simulink model "pi_rotation_loss"  (R2025b)
settings: Solver=VariableStepAuto  StartTime=0.0  StopTime=10.0  RelTol=1e-3
undefined symbols (not defined in the file): Eoff_mJ, Eon_mJ, Ic_bp, Ic_bp1, Ion, Lithium, Vce_bp
libraries: spsCurrentMeasurementLib x19, spsMosfetLib x16, simulink x16, hdlsllib x16, spsSeriesRLCBranchLib x14, spsVoltageMeasurementLib x5, spsBatteryLib x2, spsLinearTransformerLib x1, slpidlib x1, spspowerguiLib x1
(part 2 of 2)

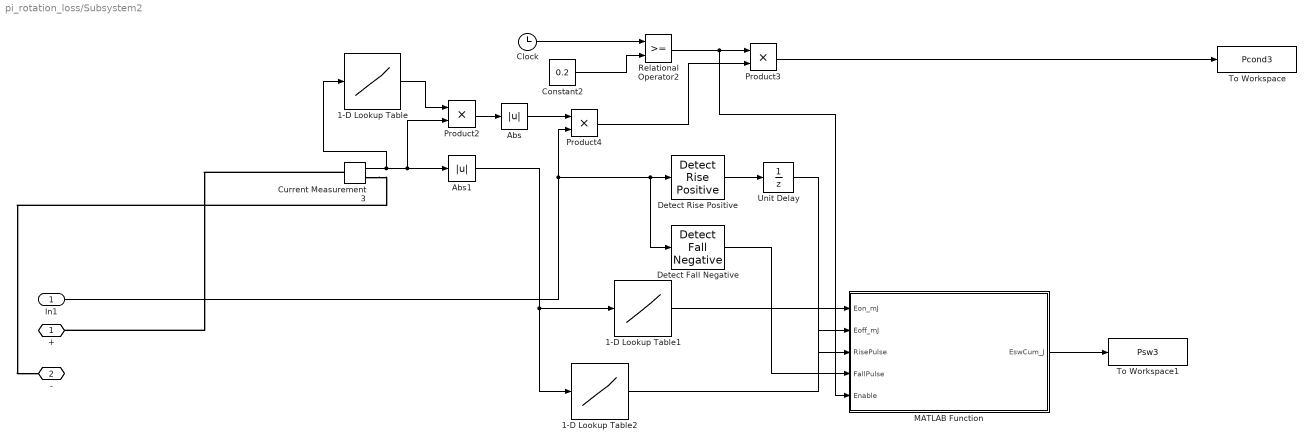
== system pi_rotation_loss/Subsystem2 ==
  In1 : Inport
  1-D Lookup Table : Lookup_n-D  NumberOfTableDimensions=1  BreakpointsForDimension1=Ic_bp  Table=Vce_bp  InternalRulePriority=Speed  RndMeth=Simplest
  1-D Lookup Table1 : Lookup_n-D  NumberOfTableDimensions=1  BreakpointsForDimension1=Ic_bp1  Table=Eon_mJ  InternalRulePriority=Speed  RndMeth=Simplest
  1-D Lookup Table2 : Lookup_n-D  NumberOfTableDimensions=1  BreakpointsForDimension1=Ic_bp1  Table=Eoff_mJ  InternalRulePriority=Speed  RndMeth=Simplest
  Abs : Abs  SaturateOnIntegerOverflow=off
  Abs1 : Abs  SaturateOnIntegerOverflow=off
  Clock : Clock
  Constant2 : Constant  Value=0.2
  Current Measurement3 : spsCurrentMeasurementLib/Current Measurement  PhasorSimulation=off  OutputType=Complex  PSBequivalent=0
  Detect Fall Negative : simulink/Logic and Bit Operations/Detect Fall Negative  vinit=0  OutDataTypeStr=boolean
  Detect Rise Positive : hdlsllib/Logic and Bit Operations/Detect Rise Positive  vinit=0  OutDataTypeStr=boolean
  MATLAB Function : MATLAB Function  TreatAsAtomicUnit=on
  Product2 : Product
  Product3 : Product
  Product4 : Product
  Relational Operator2 : RelationalOperator  OutDataTypeStr=boolean  RndMeth=Simplest  InputSameDT=off
  To Workspace : ToWorkspace  VariableName=Pcond3  SaveFormat=Timeseries  SampleTime=-1
  To Workspace1 : ToWorkspace  VariableName=Psw3  SaveFormat=Timeseries  SampleTime=-1
  Unit Delay : UnitDelay  SampleTime=-1  HasFrameUpgradeWarning=on
  + : PMIOPort  Side=Left
  - : PMIOPort  Port=2  Side=Right
  wires:
  Clock/1 -> Relational Operator2/1
  Abs/1 -> Product4/1
  Current Measurement3/1 -> Product2/2, Abs1/1, 1-D Lookup Table/1
  Unit Delay/1 -> MATLAB Function/3(RisePulse)
  1-D Lookup Table1/1 -> MATLAB Function/1(Eon_mJ)
  In1/1 -> Product4/2, Detect Fall Negative/1, Detect Rise Positive/1
  Product3/1 -> To Workspace/1
  Detect Rise Positive/1 -> Unit Delay/1
  Relational Operator2/1 -> MATLAB Function/5(Enable), Product3/1
  Product4/1 -> Product3/2
  Product2/1 -> Abs/1
  MATLAB Function/1(EswCum_J) -> To Workspace1/1
  1-D Lookup Table2/1 -> MATLAB Function/2(Eoff_mJ)
  Constant2/1 -> Relational Operator2/2
  Detect Fall Negative/1 -> MATLAB Function/4(FallPulse)
  1-D Lookup Table/1 -> Product2/1
  Abs1/1 -> 1-D Lookup Table2/1, 1-D Lookup Table1/1
  connections:
  Current Measurement3/LConn1 -- +/RConn1
  Current Measurement3/RConn1 -- -/RConn1

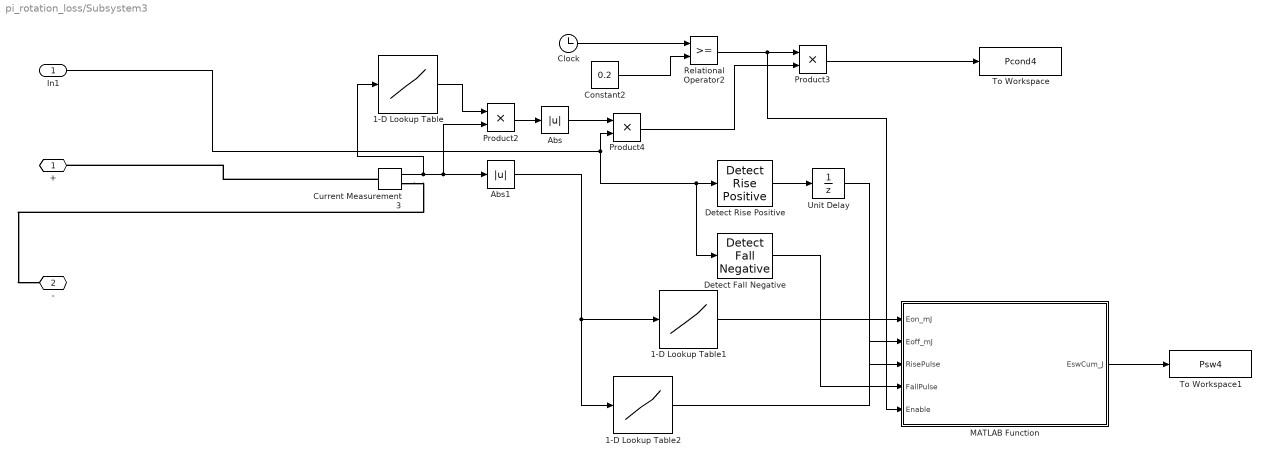
== system pi_rotation_loss/Subsystem3 ==
  In1 : Inport
  1-D Lookup Table : Lookup_n-D  NumberOfTableDimensions=1  BreakpointsForDimension1=Ic_bp  Table=Vce_bp  InternalRulePriority=Speed  RndMeth=Simplest
  1-D Lookup Table1 : Lookup_n-D  NumberOfTableDimensions=1  BreakpointsForDimension1=Ic_bp1  Table=Eon_mJ  InternalRulePriority=Speed  RndMeth=Simplest
  1-D Lookup Table2 : Lookup_n-D  NumberOfTableDimensions=1  BreakpointsForDimension1=Ic_bp1  Table=Eoff_mJ  InternalRulePriority=Speed  RndMeth=Simplest
  Abs : Abs  SaturateOnIntegerOverflow=off
  Abs1 : Abs  SaturateOnIntegerOverflow=off
  Clock : Clock
  Constant2 : Constant  Value=0.2
  Current Measurement3 : spsCurrentMeasurementLib/Current Measurement  PhasorSimulation=off  OutputType=Complex  PSBequivalent=0
  Detect Fall Negative : simulink/Logic and Bit Operations/Detect Fall Negative  vinit=0  OutDataTypeStr=boolean
  Detect Rise Positive : hdlsllib/Logic and Bit Operations/Detect Rise Positive  vinit=0  OutDataTypeStr=boolean
  MATLAB Function : MATLAB Function  TreatAsAtomicUnit=on
  Product2 : Product
  Product3 : Product
  Product4 : Product
  Relational Operator2 : RelationalOperator  OutDataTypeStr=boolean  RndMeth=Simplest  InputSameDT=off
  To Workspace : ToWorkspace  VariableName=Pcond4  SaveFormat=Timeseries  SampleTime=-1
  To Workspace1 : ToWorkspace  VariableName=Psw4  SaveFormat=Timeseries  SampleTime=-1
  Unit Delay : UnitDelay  SampleTime=-1  HasFrameUpgradeWarning=on
  + : PMIOPort  Side=Left
  - : PMIOPort  Port=2  Side=Right
  wires:
  Clock/1 -> Relational Operator2/1
  Abs/1 -> Product4/1
  Current Measurement3/1 -> Product2/2, Abs1/1, 1-D Lookup Table/1
  Unit Delay/1 -> MATLAB Function/3(RisePulse)
  1-D Lookup Table1/1 -> MATLAB Function/1(Eon_mJ)
  In1/1 -> Product4/2, Detect Fall Negative/1, Detect Rise Positive/1
  Product3/1 -> To Workspace/1
  Detect Rise Positive/1 -> Unit Delay/1
  Relational Operator2/1 -> MATLAB Function/5(Enable), Product3/1
  Product4/1 -> Product3/2
  Product2/1 -> Abs/1
  MATLAB Function/1(EswCum_J) -> To Workspace1/1
  1-D Lookup Table2/1 -> MATLAB Function/2(Eoff_mJ)
  Constant2/1 -> Relational Operator2/2
  Detect Fall Negative/1 -> MATLAB Function/4(FallPulse)
  1-D Lookup Table/1 -> Product2/1
  Abs1/1 -> 1-D Lookup Table2/1, 1-D Lookup Table1/1
  connections:
  Current Measurement3/LConn1 -- +/RConn1
  Current Measurement3/RConn1 -- -/RConn1

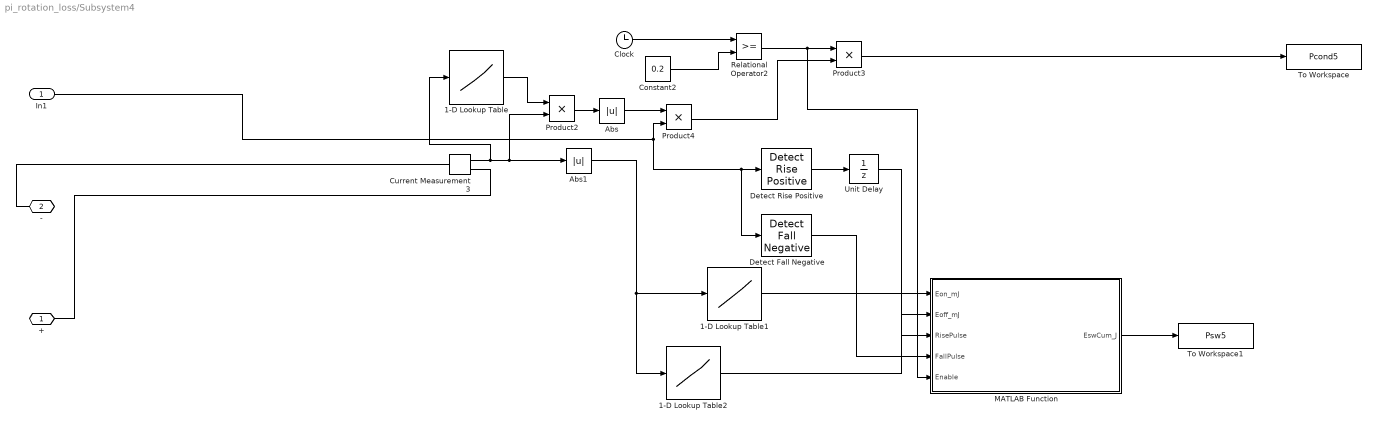
== system pi_rotation_loss/Subsystem4 ==
  In1 : Inport
  1-D Lookup Table : Lookup_n-D  NumberOfTableDimensions=1  BreakpointsForDimension1=Ic_bp  Table=Vce_bp  InternalRulePriority=Speed  RndMeth=Simplest
  1-D Lookup Table1 : Lookup_n-D  NumberOfTableDimensions=1  BreakpointsForDimension1=Ic_bp1  Table=Eon_mJ  InternalRulePriority=Speed  RndMeth=Simplest
  1-D Lookup Table2 : Lookup_n-D  NumberOfTableDimensions=1  BreakpointsForDimension1=Ic_bp1  Table=Eoff_mJ  InternalRulePriority=Speed  RndMeth=Simplest
  Abs : Abs  SaturateOnIntegerOverflow=off
  Abs1 : Abs  SaturateOnIntegerOverflow=off
  Clock : Clock
  Constant2 : Constant  Value=0.2
  Current Measurement3 : spsCurrentMeasurementLib/Current Measurement  PhasorSimulation=off  OutputType=Complex  PSBequivalent=0
  Detect Fall Negative : simulink/Logic and Bit Operations/Detect Fall Negative  vinit=0  OutDataTypeStr=boolean
  Detect Rise Positive : hdlsllib/Logic and Bit Operations/Detect Rise Positive  vinit=0  OutDataTypeStr=boolean
  MATLAB Function : MATLAB Function  TreatAsAtomicUnit=on
  Product2 : Product
  Product3 : Product
  Product4 : Product
  Relational Operator2 : RelationalOperator  OutDataTypeStr=boolean  RndMeth=Simplest  InputSameDT=off
  To Workspace : ToWorkspace  VariableName=Pcond5  SaveFormat=Timeseries  SampleTime=-1
  To Workspace1 : ToWorkspace  VariableName=Psw5  SaveFormat=Timeseries  SampleTime=-1
  Unit Delay : UnitDelay  SampleTime=-1  HasFrameUpgradeWarning=on
  + : PMIOPort  Side=Left
  - : PMIOPort  Port=2  Side=Right
  wires:
  Clock/1 -> Relational Operator2/1
  Abs/1 -> Product4/1
  Current Measurement3/1 -> Product2/2, Abs1/1, 1-D Lookup Table/1
  Unit Delay/1 -> MATLAB Function/3(RisePulse)
  1-D Lookup Table1/1 -> MATLAB Function/1(Eon_mJ)
  In1/1 -> Product4/2, Detect Fall Negative/1, Detect Rise Positive/1
  Product3/1 -> To Workspace/1
  Detect Rise Positive/1 -> Unit Delay/1
  Relational Operator2/1 -> MATLAB Function/5(Enable), Product3/1
  Product4/1 -> Product3/2
  Product2/1 -> Abs/1
  MATLAB Function/1(EswCum_J) -> To Workspace1/1
  1-D Lookup Table2/1 -> MATLAB Function/2(Eoff_mJ)
  Constant2/1 -> Relational Operator2/2
  Detect Fall Negative/1 -> MATLAB Function/4(FallPulse)
  1-D Lookup Table/1 -> Product2/1
  Abs1/1 -> 1-D Lookup Table2/1, 1-D Lookup Table1/1
  connections:
  Current Measurement3/LConn1 -- -/RConn1
  Current Measurement3/RConn1 -- +/RConn1

== system pi_rotation_loss/Subsystem5 ==
  In1 : Inport
  1-D Lookup Table : Lookup_n-D  NumberOfTableDimensions=1  BreakpointsForDimension1=Ic_bp  Table=Vce_bp  InternalRulePriority=Speed  RndMeth=Simplest
  1-D Lookup Table1 : Lookup_n-D  NumberOfTableDimensions=1  BreakpointsForDimension1=Ic_bp1  Table=Eon_mJ  InternalRulePriority=Speed  RndMeth=Simplest
  1-D Lookup Table2 : Lookup_n-D  NumberOfTableDimensions=1  BreakpointsForDimension1=Ic_bp1  Table=Eoff_mJ  InternalRulePriority=Speed  RndMeth=Simplest
  Abs : Abs  SaturateOnIntegerOverflow=off
  Abs1 : Abs  SaturateOnIntegerOverflow=off
  Clock : Clock
  Constant2 : Constant  Value=0.2
  Current Measurement3 : spsCurrentMeasurementLib/Current Measurement  PhasorSimulation=off  OutputType=Complex  PSBequivalent=0
  Detect Fall Negative : simulink/Logic and Bit Operations/Detect Fall Negative  vinit=0  OutDataTypeStr=boolean
  Detect Rise Positive : hdlsllib/Logic and Bit Operations/Detect Rise Positive  vinit=0  OutDataTypeStr=boolean
  MATLAB Function : MATLAB Function  TreatAsAtomicUnit=on
  Product2 : Product
  Product3 : Product
  Product4 : Product
  Relational Operator2 : RelationalOperator  OutDataTypeStr=boolean  RndMeth=Simplest  InputSameDT=off
  To Workspace : ToWorkspace  VariableName=Pcond6  SaveFormat=Timeseries  SampleTime=-1
  To Workspace1 : ToWorkspace  VariableName=Psw6  SaveFormat=Timeseries  SampleTime=-1
  Unit Delay : UnitDelay  SampleTime=-1  HasFrameUpgradeWarning=on
  + : PMIOPort  Side=Left
  - : PMIOPort  Port=2  Side=Right
  wires:
  Clock/1 -> Relational Operator2/1
  Abs/1 -> Product4/1
  Current Measurement3/1 -> Product2/2, Abs1/1, 1-D Lookup Table/1
  Unit Delay/1 -> MATLAB Function/3(RisePulse)
  1-D Lookup Table1/1 -> MATLAB Function/1(Eon_mJ)
  In1/1 -> Product4/2, Detect Fall Negative/1, Detect Rise Positive/1
  Product3/1 -> To Workspace/1
  Detect Rise Positive/1 -> Unit Delay/1
  Relational Operator2/1 -> MATLAB Function/5(Enable), Product3/1
  Product4/1 -> Product3/2
  Product2/1 -> Abs/1
  MATLAB Function/1(EswCum_J) -> To Workspace1/1
  1-D Lookup Table2/1 -> MATLAB Function/2(Eoff_mJ)
  Constant2/1 -> Relational Operator2/2
  Detect Fall Negative/1 -> MATLAB Function/4(FallPulse)
  1-D Lookup Table/1 -> Product2/1
  Abs1/1 -> 1-D Lookup Table2/1, 1-D Lookup Table1/1
  connections:
  Current Measurement3/LConn1 -- +/RConn1
  Current Measurement3/RConn1 -- -/RConn1

== system pi_rotation_loss/Subsystem6 ==
  In1 : Inport
  1-D Lookup Table : Lookup_n-D  NumberOfTableDimensions=1  BreakpointsForDimension1=Ic_bp  Table=Vce_bp  InternalRulePriority=Speed  RndMeth=Simplest
  1-D Lookup Table1 : Lookup_n-D  NumberOfTableDimensions=1  BreakpointsForDimension1=Ic_bp1  Table=Eon_mJ  InternalRulePriority=Speed  RndMeth=Simplest
  1-D Lookup Table2 : Lookup_n-D  NumberOfTableDimensions=1  BreakpointsForDimension1=Ic_bp1  Table=Eoff_mJ  InternalRulePriority=Speed  RndMeth=Simplest
  Abs : Abs  SaturateOnIntegerOverflow=off
  Abs1 : Abs  SaturateOnIntegerOverflow=off
  Clock : Clock
  Constant2 : Constant  Value=0.2
  Current Measurement3 : spsCurrentMeasurementLib/Current Measurement  PhasorSimulation=off  OutputType=Complex  PSBequivalent=0
  Detect Fall Negative : simulink/Logic and Bit Operations/Detect Fall Negative  vinit=0  OutDataTypeStr=boolean
  Detect Rise Positive : hdlsllib/Logic and Bit Operations/Detect Rise Positive  vinit=0  OutDataTypeStr=boolean
  MATLAB Function : MATLAB Function  TreatAsAtomicUnit=on
  Product2 : Product
  Product3 : Product
  Product4 : Product
  Relational Operator2 : RelationalOperator  OutDataTypeStr=boolean  RndMeth=Simplest  InputSameDT=off
  To Workspace : ToWorkspace  VariableName=Pcond8  SaveFormat=Timeseries  SampleTime=-1
  To Workspace1 : ToWorkspace  VariableName=Psw8  SaveFormat=Timeseries  SampleTime=-1
  Unit Delay : UnitDelay  SampleTime=-1  HasFrameUpgradeWarning=on
  + : PMIOPort  Side=Left
  - : PMIOPort  Port=2  Side=Right
  wires:
  Clock/1 -> Relational Operator2/1
  Abs/1 -> Product4/1
  Current Measurement3/1 -> Product2/2, Abs1/1, 1-D Lookup Table/1
  Unit Delay/1 -> MATLAB Function/3(RisePulse)
  1-D Lookup Table1/1 -> MATLAB Function/1(Eon_mJ)
  In1/1 -> Product4/2, Detect Fall Negative/1, Detect Rise Positive/1
  Product3/1 -> To Workspace/1
  Detect Rise Positive/1 -> Unit Delay/1
  Relational Operator2/1 -> MATLAB Function/5(Enable), Product3/1
  Product4/1 -> Product3/2
  Product2/1 -> Abs/1
  MATLAB Function/1(EswCum_J) -> To Workspace1/1
  1-D Lookup Table2/1 -> MATLAB Function/2(Eoff_mJ)
  Constant2/1 -> Relational Operator2/2
  Detect Fall Negative/1 -> MATLAB Function/4(FallPulse)
  1-D Lookup Table/1 -> Product2/1
  Abs1/1 -> 1-D Lookup Table2/1, 1-D Lookup Table1/1
  connections:
  Current Measurement3/LConn1 -- +/RConn1
  Current Measurement3/RConn1 -- -/RConn1

== system pi_rotation_loss/Subsystem7 ==
  In1 : Inport
  1-D Lookup Table : Lookup_n-D  NumberOfTableDimensions=1  BreakpointsForDimension1=Ic_bp  Table=Vce_bp  InternalRulePriority=Speed  RndMeth=Simplest
  1-D Lookup Table1 : Lookup_n-D  NumberOfTableDimensions=1  BreakpointsForDimension1=Ic_bp1  Table=Eon_mJ  InternalRulePriority=Speed  RndMeth=Simplest
  1-D Lookup Table2 : Lookup_n-D  NumberOfTableDimensions=1  BreakpointsForDimension1=Ic_bp1  Table=Eoff_mJ  InternalRulePriority=Speed  RndMeth=Simplest
  Abs : Abs  SaturateOnIntegerOverflow=off
  Abs1 : Abs  SaturateOnIntegerOverflow=off
  Clock : Clock
  Constant2 : Constant  Value=0.2
  Current Measurement3 : spsCurrentMeasurementLib/Current Measurement  PhasorSimulation=off  OutputType=Complex  PSBequivalent=0
  Detect Fall Negative : simulink/Logic and Bit Operations/Detect Fall Negative  vinit=0  OutDataTypeStr=boolean
  Detect Rise Positive : hdlsllib/Logic and Bit Operations/Detect Rise Positive  vinit=0  OutDataTypeStr=boolean
  MATLAB Function : MATLAB Function  TreatAsAtomicUnit=on
  Product2 : Product
  Product3 : Product
  Product4 : Product
  Relational Operator2 : RelationalOperator  OutDataTypeStr=boolean  RndMeth=Simplest  InputSameDT=off
  To Workspace : ToWorkspace  VariableName=Pcond7  SaveFormat=Timeseries  SampleTime=-1
  To Workspace1 : ToWorkspace  VariableName=Psw7  SaveFormat=Timeseries  SampleTime=-1
  Unit Delay : UnitDelay  SampleTime=-1  HasFrameUpgradeWarning=on
  + : PMIOPort  Side=Left
  - : PMIOPort  Port=2  Side=Right
  wires:
  Clock/1 -> Relational Operator2/1
  Abs/1 -> Product4/1
  Current Measurement3/1 -> Product2/2, Abs1/1, 1-D Lookup Table/1
  Unit Delay/1 -> MATLAB Function/3(RisePulse)
  1-D Lookup Table1/1 -> MATLAB Function/1(Eon_mJ)
  In1/1 -> Product4/2, Detect Fall Negative/1, Detect Rise Positive/1
  Product3/1 -> To Workspace/1
  Detect Rise Positive/1 -> Unit Delay/1
  Relational Operator2/1 -> MATLAB Function/5(Enable), Product3/1
  Product4/1 -> Product3/2
  Product2/1 -> Abs/1
  MATLAB Function/1(EswCum_J) -> To Workspace1/1
  1-D Lookup Table2/1 -> MATLAB Function/2(Eoff_mJ)
  Constant2/1 -> Relational Operator2/2
  Detect Fall Negative/1 -> MATLAB Function/4(FallPulse)
  1-D Lookup Table/1 -> Product2/1
  Abs1/1 -> 1-D Lookup Table2/1, 1-D Lookup Table1/1
  connections:
  Current Measurement3/LConn1 -- +/RConn1
  Current Measurement3/RConn1 -- -/RConn1

== system pi_rotation_loss/Subsystem8 ==
  In1 : Inport
  1-D Lookup Table : Lookup_n-D  NumberOfTableDimensions=1  BreakpointsForDimension1=Ic_bp  Table=Vce_bp  InternalRulePriority=Speed  RndMeth=Simplest
  1-D Lookup Table1 : Lookup_n-D  NumberOfTableDimensions=1  BreakpointsForDimension1=Ic_bp1  Table=Eon_mJ  InternalRulePriority=Speed  RndMeth=Simplest
  1-D Lookup Table2 : Lookup_n-D  NumberOfTableDimensions=1  BreakpointsForDimension1=Ic_bp1  Table=Eoff_mJ  InternalRulePriority=Speed  RndMeth=Simplest
  Abs : Abs  SaturateOnIntegerOverflow=off
  Abs1 : Abs  SaturateOnIntegerOverflow=off
  Clock : Clock
  Constant2 : Constant  Value=0.2
  Current Measurement3 : spsCurrentMeasurementLib/Current Measurement  PhasorSimulation=off  OutputType=Complex  PSBequivalent=0
  Detect Fall Negative : simulink/Logic and Bit Operations/Detect Fall Negative  vinit=0  OutDataTypeStr=boolean
  Detect Rise Positive : hdlsllib/Logic and Bit Operations/Detect Rise Positive  vinit=0  OutDataTypeStr=boolean
  MATLAB Function : MATLAB Function  TreatAsAtomicUnit=on
  Product2 : Product
  Product3 : Product
  Product4 : Product
  Relational Operator2 : RelationalOperator  OutDataTypeStr=boolean  RndMeth=Simplest  InputSameDT=off
  To Workspace : ToWorkspace  VariableName=Pcond7_2  SaveFormat=Timeseries  SampleTime=-1
  To Workspace1 : ToWorkspace  VariableName=Psw7_2  SaveFormat=Timeseries  SampleTime=-1
  Unit Delay : UnitDelay  SampleTime=-1  HasFrameUpgradeWarning=on
  + : PMIOPort  Side=Left
  - : PMIOPort  Port=2  Side=Right
  wires:
  Clock/1 -> Relational Operator2/1
  Abs/1 -> Product4/1
  Current Measurement3/1 -> Product2/2, Abs1/1, 1-D Lookup Table/1
  Unit Delay/1 -> MATLAB Function/3(RisePulse)
  1-D Lookup Table1/1 -> MATLAB Function/1(Eon_mJ)
  In1/1 -> Product4/2, Detect Fall Negative/1, Detect Rise Positive/1
  Product3/1 -> To Workspace/1
  Detect Rise Positive/1 -> Unit Delay/1
  Relational Operator2/1 -> MATLAB Function/5(Enable), Product3/1
  Product4/1 -> Product3/2
  Product2/1 -> Abs/1
  MATLAB Function/1(EswCum_J) -> To Workspace1/1
  1-D Lookup Table2/1 -> MATLAB Function/2(Eoff_mJ)
  Constant2/1 -> Relational Operator2/2
  Detect Fall Negative/1 -> MATLAB Function/4(FallPulse)
  1-D Lookup Table/1 -> Product2/1
  Abs1/1 -> 1-D Lookup Table2/1, 1-D Lookup Table1/1
  connections:
  Current Measurement3/LConn1 -- +/RConn1
  Current Measurement3/RConn1 -- -/RConn1

== system pi_rotation_loss/Subsystem9 ==
  In1 : Inport
  1-D Lookup Table : Lookup_n-D  NumberOfTableDimensions=1  BreakpointsForDimension1=Ic_bp  Table=Vce_bp  InternalRulePriority=Speed  RndMeth=Simplest
  1-D Lookup Table1 : Lookup_n-D  NumberOfTableDimensions=1  BreakpointsForDimension1=Ic_bp1  Table=Eon_mJ  InternalRulePriority=Speed  RndMeth=Simplest
  1-D Lookup Table2 : Lookup_n-D  NumberOfTableDimensions=1  BreakpointsForDimension1=Ic_bp1  Table=Eoff_mJ  InternalRulePriority=Speed  RndMeth=Simplest
  Abs : Abs  SaturateOnIntegerOverflow=off
  Abs1 : Abs  SaturateOnIntegerOverflow=off
  Clock : Clock
  Constant2 : Constant  Value=0.2
  Current Measurement3 : spsCurrentMeasurementLib/Current Measurement  PhasorSimulation=off  OutputType=Complex  PSBequivalent=0
  Detect Fall Negative : simulink/Logic and Bit Operations/Detect Fall Negative  vinit=0  OutDataTypeStr=boolean
  Detect Rise Positive : hdlsllib/Logic and Bit Operations/Detect Rise Positive  vinit=0  OutDataTypeStr=boolean
  MATLAB Function : MATLAB Function  TreatAsAtomicUnit=on
  Product2 : Product
  Product3 : Product
  Product4 : Product
  Relational Operator2 : RelationalOperator  OutDataTypeStr=boolean  RndMeth=Simplest  InputSameDT=off
  To Workspace : ToWorkspace  VariableName=Pcond8_2  SaveFormat=Timeseries  SampleTime=-1
  To Workspace1 : ToWorkspace  VariableName=Psw8_2  SaveFormat=Timeseries  SampleTime=-1
  Unit Delay : UnitDelay  SampleTime=-1  HasFrameUpgradeWarning=on
  + : PMIOPort  Side=Left
  - : PMIOPort  Port=2  Side=Right
  wires:
  Clock/1 -> Relational Operator2/1
  Abs/1 -> Product4/1
  Current Measurement3/1 -> Product2/2, Abs1/1, 1-D Lookup Table/1
  Unit Delay/1 -> MATLAB Function/3(RisePulse)
  1-D Lookup Table1/1 -> MATLAB Function/1(Eon_mJ)
  In1/1 -> Product4/2, Detect Fall Negative/1, Detect Rise Positive/1
  Product3/1 -> To Workspace/1
  Detect Rise Positive/1 -> Unit Delay/1
  Relational Operator2/1 -> MATLAB Function/5(Enable), Product3/1
  Product4/1 -> Product3/2
  Product2/1 -> Abs/1
  MATLAB Function/1(EswCum_J) -> To Workspace1/1
  1-D Lookup Table2/1 -> MATLAB Function/2(Eoff_mJ)
  Constant2/1 -> Relational Operator2/2
  Detect Fall Negative/1 -> MATLAB Function/4(FallPulse)
  1-D Lookup Table/1 -> Product2/1
  Abs1/1 -> 1-D Lookup Table2/1, 1-D Lookup Table1/1
  connections:
  Current Measurement3/LConn1 -- +/RConn1
  Current Measurement3/RConn1 -- -/RConn1

== matlab function pi_rotation_loss/Subsystem15/MATLAB Function ==
  data: Eon_mJ input; EswCum_J output; Eoff_mJ input; RisePulse input; FallPulse input; Enable input
function EswCum_J = accumulate_energy( ...
    Eon_mJ, Eoff_mJ, RisePulse, FallPulse, Enable)
%#codegen
% Eon_mJ and Eoff_mJ are lookup outputs in millijoules.
% Output EswCum_J is cumulative switching energy in joules.
% Accumulate only events occurring after t = 0.2 s.

persistent cumulative_J

if isempty(cumulative_J)
    cumulative_J = 0.0;
end

if Enable > 0.5

    if RisePulse > 0.5
        cumulative_J = cumulative_J + max(Eon_mJ, 0) * 1e-3;
    end

    if FallPulse > 0.5
        cumulative_J = cumulative_J + max(Eoff_mJ, 0) * 1e-3;
    end

end

EswCum_J = cumulative_J;
end

== matlab function pi_rotation_loss/Subsystem/MATLAB Function ==
  data: Eon_mJ input; EswCum_J output; Eoff_mJ input; RisePulse input; FallPulse input; Enable input
function EswCum_J = accumulate_energy( ...
    Eon_mJ, Eoff_mJ, RisePulse, FallPulse, Enable)
%#codegen
% Eon_mJ and Eoff_mJ are lookup outputs in millijoules.
% Output EswCum_J is cumulative switching energy in joules.
% Accumulate only events occurring after t = 0.2 s.

persistent cumulative_J

if isempty(cumulative_J)
    cumulative_J = 0.0;
end

if Enable > 0.5

    if RisePulse > 0.5
        cumulative_J = cumulative_J + max(Eon_mJ, 0) * 1e-3;
    end

    if FallPulse > 0.5
        cumulative_J = cumulative_J + max(Eoff_mJ, 0) * 1e-3;
    end

end

EswCum_J = cumulative_J;
end

== matlab function pi_rotation_loss/Subsystem12/MATLAB Function ==
  data: Eon_mJ input; EswCum_J output; Eoff_mJ input; RisePulse input; FallPulse input; Enable input
function EswCum_J = accumulate_energy( ...
    Eon_mJ, Eoff_mJ, RisePulse, FallPulse, Enable)
%#codegen
% Eon_mJ and Eoff_mJ are lookup outputs in millijoules.
% Output EswCum_J is cumulative switching energy in joules.
% Accumulate only events occurring after t = 0.2 s.

persistent cumulative_J

if isempty(cumulative_J)
    cumulative_J = 0.0;
end

if Enable > 0.5

    if RisePulse > 0.5
        cumulative_J = cumulative_J + max(Eon_mJ, 0) * 1e-3;
    end

    if FallPulse > 0.5
        cumulative_J = cumulative_J + max(Eoff_mJ, 0) * 1e-3;
    end

end

EswCum_J = cumulative_J;
end

== matlab function pi_rotation_loss/Subsystem14/MATLAB Function ==
  data: Eon_mJ input; EswCum_J output; Eoff_mJ input; RisePulse input; FallPulse input; Enable input
function EswCum_J = accumulate_energy( ...
    Eon_mJ, Eoff_mJ, RisePulse, FallPulse, Enable)
%#codegen
% Eon_mJ and Eoff_mJ are lookup outputs in millijoules.
% Output EswCum_J is cumulative switching energy in joules.
% Accumulate only events occurring after t = 0.2 s.

persistent cumulative_J

if isempty(cumulative_J)
    cumulative_J = 0.0;
end

if Enable > 0.5

    if RisePulse > 0.5
        cumulative_J = cumulative_J + max(Eon_mJ, 0) * 1e-3;
    end

    if FallPulse > 0.5
        cumulative_J = cumulative_J + max(Eoff_mJ, 0) * 1e-3;
    end

end

EswCum_J = cumulative_J;
end

== matlab function pi_rotation_loss/Subsystem11/MATLAB Function ==
  data: Eon_mJ input; EswCum_J output; Eoff_mJ input; RisePulse input; FallPulse input; Enable input
function EswCum_J = accumulate_energy( ...
    Eon_mJ, Eoff_mJ, RisePulse, FallPulse, Enable)
%#codegen
% Eon_mJ and Eoff_mJ are lookup outputs in millijoules.
% Output EswCum_J is cumulative switching energy in joules.
% Accumulate only events occurring after t = 0.2 s.

persistent cumulative_J

if isempty(cumulative_J)
    cumulative_J = 0.0;
end

if Enable > 0.5

    if RisePulse > 0.5
        cumulative_J = cumulative_J + max(Eon_mJ, 0) * 1e-3;
    end

    if FallPulse > 0.5
        cumulative_J = cumulative_J + max(Eoff_mJ, 0) * 1e-3;
    end

end

EswCum_J = cumulative_J;
end

== matlab function pi_rotation_loss/Subsystem13/MATLAB Function ==
  data: Eon_mJ input; EswCum_J output; Eoff_mJ input; RisePulse input; FallPulse input; Enable input
function EswCum_J = accumulate_energy( ...
    Eon_mJ, Eoff_mJ, RisePulse, FallPulse, Enable)
%#codegen
% Eon_mJ and Eoff_mJ are lookup outputs in millijoules.
% Output EswCum_J is cumulative switching energy in joules.
% Accumulate only events occurring after t = 0.2 s.

persistent cumulative_J

if isempty(cumulative_J)
    cumulative_J = 0.0;
end

if Enable > 0.5

    if RisePulse > 0.5
        cumulative_J = cumulative_J + max(Eon_mJ, 0) * 1e-3;
    end

    if FallPulse > 0.5
        cumulative_J = cumulative_J + max(Eoff_mJ, 0) * 1e-3;
    end

end

EswCum_J = cumulative_J;
end

== matlab function pi_rotation_loss/Subsystem10/MATLAB Function ==
  data: Eon_mJ input; EswCum_J output; Eoff_mJ input; RisePulse input; FallPulse input; Enable input
function EswCum_J = accumulate_energy( ...
    Eon_mJ, Eoff_mJ, RisePulse, FallPulse, Enable)
%#codegen
% Eon_mJ and Eoff_mJ are lookup outputs in millijoules.
% Output EswCum_J is cumulative switching energy in joules.
% Accumulate only events occurring after t = 0.2 s.

persistent cumulative_J

if isempty(cumulative_J)
    cumulative_J = 0.0;
end

if Enable > 0.5

    if RisePulse > 0.5
        cumulative_J = cumulative_J + max(Eon_mJ, 0) * 1e-3;
    end

    if FallPulse > 0.5
        cumulative_J = cumulative_J + max(Eoff_mJ, 0) * 1e-3;
    end

end

EswCum_J = cumulative_J;
end

== matlab function pi_rotation_loss/Subsystem9/MATLAB Function ==
  data: Eon_mJ input; EswCum_J output; Eoff_mJ input; RisePulse input; FallPulse input; Enable input
function EswCum_J = accumulate_energy( ...
    Eon_mJ, Eoff_mJ, RisePulse, FallPulse, Enable)
%#codegen
% Eon_mJ and Eoff_mJ are lookup outputs in millijoules.
% Output EswCum_J is cumulative switching energy in joules.
% Accumulate only events occurring after t = 0.2 s.

persistent cumulative_J

if isempty(cumulative_J)
    cumulative_J = 0.0;
end

if Enable > 0.5

    if RisePulse > 0.5
        cumulative_J = cumulative_J + max(Eon_mJ, 0) * 1e-3;
    end

    if FallPulse > 0.5
        cumulative_J = cumulative_J + max(Eoff_mJ, 0) * 1e-3;
    end

end

EswCum_J = cumulative_J;
end

== matlab function pi_rotation_loss/Subsystem8/MATLAB Function ==
  data: Eon_mJ input; EswCum_J output; Eoff_mJ input; RisePulse input; FallPulse input; Enable input
function EswCum_J = accumulate_energy( ...
    Eon_mJ, Eoff_mJ, RisePulse, FallPulse, Enable)
%#codegen
% Eon_mJ and Eoff_mJ are lookup outputs in millijoules.
% Output EswCum_J is cumulative switching energy in joules.
% Accumulate only events occurring after t = 0.2 s.

persistent cumulative_J

if isempty(cumulative_J)
    cumulative_J = 0.0;
end

if Enable > 0.5

    if RisePulse > 0.5
        cumulative_J = cumulative_J + max(Eon_mJ, 0) * 1e-3;
    end

    if FallPulse > 0.5
        cumulative_J = cumulative_J + max(Eoff_mJ, 0) * 1e-3;
    end

end

EswCum_J = cumulative_J;
end

== matlab function pi_rotation_loss/MATLAB Function ==
  data: t input; y output
function y = fcn(t)

f = 20000;      % 20 kHz
T = 1/f;

x = mod(t,T)/T;

if x < 0.5
    y = 2*x;
else
    y = 2*(1-x);
end

end

== matlab function pi_rotation_loss/Subsystem1/MATLAB Function ==
  data: Eon_mJ input; EswCum_J output; Eoff_mJ input; RisePulse input; FallPulse input; Enable input
function EswCum_J = accumulate_energy( ...
    Eon_mJ, Eoff_mJ, RisePulse, FallPulse, Enable)
%#codegen
% Eon_mJ and Eoff_mJ are lookup outputs in millijoules.
% Output EswCum_J is cumulative switching energy in joules.
% Accumulate only events occurring after t = 0.2 s.

persistent cumulative_J

if isempty(cumulative_J)
    cumulative_J = 0.0;
end

if Enable > 0.5

    if RisePulse > 0.5
        cumulative_J = cumulative_J + max(Eon_mJ, 0) * 1e-3;
    end

    if FallPulse > 0.5
        cumulative_J = cumulative_J + max(Eoff_mJ, 0) * 1e-3;
    end

end

EswCum_J = cumulative_J;
end

== matlab function pi_rotation_loss/Subsystem3/MATLAB Function ==
  data: Eon_mJ input; EswCum_J output; Eoff_mJ input; RisePulse input; FallPulse input; Enable input
function EswCum_J = accumulate_energy( ...
    Eon_mJ, Eoff_mJ, RisePulse, FallPulse, Enable)
%#codegen
% Eon_mJ and Eoff_mJ are lookup outputs in millijoules.
% Output EswCum_J is cumulative switching energy in joules.
% Accumulate only events occurring after t = 0.2 s.

persistent cumulative_J

if isempty(cumulative_J)
    cumulative_J = 0.0;
end

if Enable > 0.5

    if RisePulse > 0.5
        cumulative_J = cumulative_J + max(Eon_mJ, 0) * 1e-3;
    end

    if FallPulse > 0.5
        cumulative_J = cumulative_J + max(Eoff_mJ, 0) * 1e-3;
    end

end

EswCum_J = cumulative_J;
end

== matlab function pi_rotation_loss/Subsystem2/MATLAB Function ==
  data: Eon_mJ input; EswCum_J output; Eoff_mJ input; RisePulse input; FallPulse input; Enable input
function EswCum_J = accumulate_energy( ...
    Eon_mJ, Eoff_mJ, RisePulse, FallPulse, Enable)
%#codegen
% Eon_mJ and Eoff_mJ are lookup outputs in millijoules.
% Output EswCum_J is cumulative switching energy in joules.
% Accumulate only events occurring after t = 0.2 s.

persistent cumulative_J

if isempty(cumulative_J)
    cumulative_J = 0.0;
end

if Enable > 0.5

    if RisePulse > 0.5
        cumulative_J = cumulative_J + max(Eon_mJ, 0) * 1e-3;
    end

    if FallPulse > 0.5
        cumulative_J = cumulative_J + max(Eoff_mJ, 0) * 1e-3;
    end

end

EswCum_J = cumulative_J;
end

== matlab function pi_rotation_loss/Subsystem4/MATLAB Function ==
  data: Eon_mJ input; EswCum_J output; Eoff_mJ input; RisePulse input; FallPulse input; Enable input
function EswCum_J = accumulate_energy( ...
    Eon_mJ, Eoff_mJ, RisePulse, FallPulse, Enable)
%#codegen
% Eon_mJ and Eoff_mJ are lookup outputs in millijoules.
% Output EswCum_J is cumulative switching energy in joules.
% Accumulate only events occurring after t = 0.2 s.

persistent cumulative_J

if isempty(cumulative_J)
    cumulative_J = 0.0;
end

if Enable > 0.5

    if RisePulse > 0.5
        cumulative_J = cumulative_J + max(Eon_mJ, 0) * 1e-3;
    end

    if FallPulse > 0.5
        cumulative_J = cumulative_J + max(Eoff_mJ, 0) * 1e-3;
    end

end

EswCum_J = cumulative_J;
end

== matlab function pi_rotation_loss/Subsystem5/MATLAB Function ==
  data: Eon_mJ input; EswCum_J output; Eoff_mJ input; RisePulse input; FallPulse input; Enable input
function EswCum_J = accumulate_energy( ...
    Eon_mJ, Eoff_mJ, RisePulse, FallPulse, Enable)
%#codegen
% Eon_mJ and Eoff_mJ are lookup outputs in millijoules.
% Output EswCum_J is cumulative switching energy in joules.
% Accumulate only events occurring after t = 0.2 s.

persistent cumulative_J

if isempty(cumulative_J)
    cumulative_J = 0.0;
end

if Enable > 0.5

    if RisePulse > 0.5
        cumulative_J = cumulative_J + max(Eon_mJ, 0) * 1e-3;
    end

    if FallPulse > 0.5
        cumulative_J = cumulative_J + max(Eoff_mJ, 0) * 1e-3;
    end

end

EswCum_J = cumulative_J;
end

== matlab function pi_rotation_loss/Subsystem7/MATLAB Function ==
  data: Eon_mJ input; EswCum_J output; Eoff_mJ input; RisePulse input; FallPulse input; Enable input
function EswCum_J = accumulate_energy( ...
    Eon_mJ, Eoff_mJ, RisePulse, FallPulse, Enable)
%#codegen
% Eon_mJ and Eoff_mJ are lookup outputs in millijoules.
% Output EswCum_J is cumulative switching energy in joules.
% Accumulate only events occurring after t = 0.2 s.

persistent cumulative_J

if isempty(cumulative_J)
    cumulative_J = 0.0;
end

if Enable > 0.5

    if RisePulse > 0.5
        cumulative_J = cumulative_J + max(Eon_mJ, 0) * 1e-3;
    end

    if FallPulse > 0.5
        cumulative_J = cumulative_J + max(Eoff_mJ, 0) * 1e-3;
    end

end

EswCum_J = cumulative_J;
end

== matlab function pi_rotation_loss/Subsystem6/MATLAB Function ==
  data: Eon_mJ input; EswCum_J output; Eoff_mJ input; RisePulse input; FallPulse input; Enable input
function EswCum_J = accumulate_energy( ...
    Eon_mJ, Eoff_mJ, RisePulse, FallPulse, Enable)
%#codegen
% Eon_mJ and Eoff_mJ are lookup outputs in millijoules.
% Output EswCum_J is cumulative switching energy in joules.
% Accumulate only events occurring after t = 0.2 s.

persistent cumulative_J

if isempty(cumulative_J)
    cumulative_J = 0.0;
end

if Enable > 0.5

    if RisePulse > 0.5
        cumulative_J = cumulative_J + max(Eon_mJ, 0) * 1e-3;
    end

    if FallPulse > 0.5
        cumulative_J = cumulative_J + max(Eoff_mJ, 0) * 1e-3;
    end

end

EswCum_J = cumulative_J;
end
